simulink model "ssc_hydraulic_lift_LibLinks"  (R2025a)
settings: Solver=ode23t  StartTime=0.0  StopTime=20  MaxStep=0.02  RelTol=1e-3  AbsTol=1e-4  EnableMultiTasking=on
PreLoadFcn:
  | warning('off','Simulink:Commands:LoadMdlParameterizedLink');
PostLoadFcn:
  | warning off sm:compiler:topologyAnalysis:DanglingBlock
  | warning off Simulink:SL_SolverMaskedZC;
  | warning off Simulink:SL_SolverIgnoredZCBracketing;
  | warning off Simulink:Engine:SolverMinStepNonlinearIterWarnForDAE;
  | warning off simscape:compiler:sli:init:SolverNotRecommended
  | warning off Simulink:Engine:UsingDiscreteSolver
  | warning('off','sm:sli:setup:compile:LocalSolverNotSupported')
  | warning off physmod:simscape:compiler:sli:init:SolverNotRecommended
  | warning off sm:sli:visualization:ModelRefNotSupported
  | warning off Simulink:modelReference:ProtectedModelCallbackLostWarning
  | 
  | load_system('Cylinder_Lib');
  | load_system('Motor_Lib');
  | load_system('Valve_Lib');
  | load_system('Load_Lib');
StartFcn:
  | tic;
StopFcn:
  | Elapsed_Sim_Time = toc;
  | disp(['Elapsed Sim Time = ' num2str(Elapsed_Sim_Time)]);
undefined symbols (not defined in the file or in its folder): Scissor_Lift_Param, sigbuilder_block
libraries: fl_lib x4, nesl_utility x4, Cylinder_Lib x2, Controller_Lib x2, Load_Lib x2, Motor_Lib x2, Valve_Lib x2
Description:
  | Copyright 2015-2025 The MathWorks, Inc.
settings Model: ExtModeTrigDuration=500  Creator=smiller  LastModifiedBy=smiller
settings SolverCC: AutoScaleAbsTol=off  ConcurrentTasks=on  AlgebraicLoopSolver=TrustRegion  PositivePriorityOrder=on
settings DataIOCC: SaveFormat=Array  ReturnWorkspaceOutputs=off
settings OptimizationCC: BlockReduction=off  OptimizeBlockIOStorage=off  BufferReuse=off  ReuseModelBlockBuffer=off  GlobalBufferReuse=off  ExpressionFolding=off  ExpressionDepthLimit=2147483647.0  LocalBlockOutputs=off  ZeroExternalMemoryAtStartup=off  ZeroInternalMemoryAtStartup=off  OptimizeDataStoreBuffers=off  BusAssignmentInplaceUpdate=off
settings DebuggingCC: UnderspecifiedInitializationDetection=Classic  MergeDetectMultiDrivingBlocksExec=none  UnconnectedInputMsg=warning  UnconnectedOutputMsg=warning  UnconnectedLineMsg=warning  AllowSymbolicDim=off  StateNameClashWarn=warning  PregeneratedLibrarySubsystemCodeDiagnostic=none  SFUnexpectedBacktrackingDiag=warning  SFNoUnconditionalDefaultTransitionDiag=warning  SFExecutionAtInitializationDiag=none  ArithmeticOperatorsInVariantConditions=warning
settings ModelReferenceCC: EnableRefExpFcnMdlSchedulingChecks=on  PropagateSignalLabelsOutOfModel=off
settings SFSimCC: SimUseLocalCustomCode=off  CustomCodeUndefinedFunction=UseInterfaceOnly
settings RTWCC: RTWUseLocalCustomCode=off  Toolchain=Simulink Real-Time Toolchain  BuildConfiguration=Faster Runs  TargetLang=C++  GPUComputeCapability=3.5  DLArmComputeVersion=19.05
settings CodeAppCC: StateflowObjectComments=on
settings GRTTargetCC: TargetLangStandard=C++03 (ISO)  CodeInterfacePackaging=C++ class
settings ConfigComp: CovMetricSettings=dw  CovSaveCumulativeToWorkspaceVar=on  CovSaveSingleToWorkspaceVar=on  CovExternalEMLEnable=off  CovSFcnEnable=off
settings SimscapeCC: ExplicitSolverDiagnosticOptions=none  SimscapeNormalizeSystem=off  SimscapeNominalValues="[{\"value\":\"10\",\"unit\":\"V\"},{\"value\":\"1\",\"unit\":\"A\"},{\"value\":\"10\",\"unit\":\"N*m\"},{\"value\":\"10\",\"unit\":\"bar\"},{\"value\":\"100\",\"unit\":\"kJ/kg\"},{\"value\":\"1\",\"unit\":\"kW\"},{\"value\":\"300\",\"unit\":\"K\"},{\"value\":\"100\",\"unit\":\"cm^3/s\"},{\"value\":\"1\",\"unit\":\"kN\"},{\"value\":\"1\",\"unit\":\"g/cm^3\"},{\"value\":\"1\",\"unit\":\"l\"},{\"value\":\"1\",\"unit\":\"cm^2\"},{\"value\":\"60\",\"unit\":\"Hz\"}]"  SimscapeLogType=all  SimscapeLogSimulationStatistics=on  SimscapeLogName=simlog_ssc_hydraulic_lift  SimscapeLogLimitData=off
settings DiagnosticsConfigSet: SimMechanicsUnconnectedFramePorts=none  SimMechanicsConflictingReferenceFrames=none

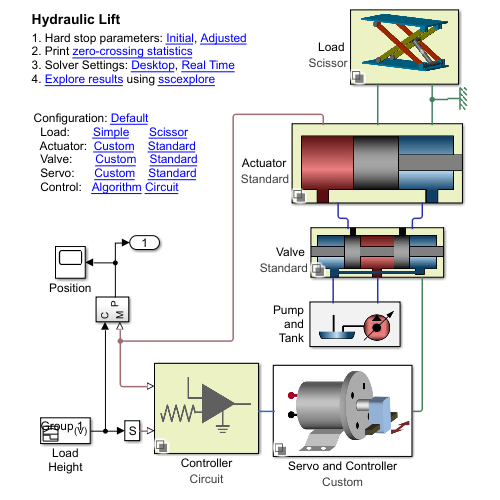
[thumbnail: Simulink's stored preview of the top-level diagram]
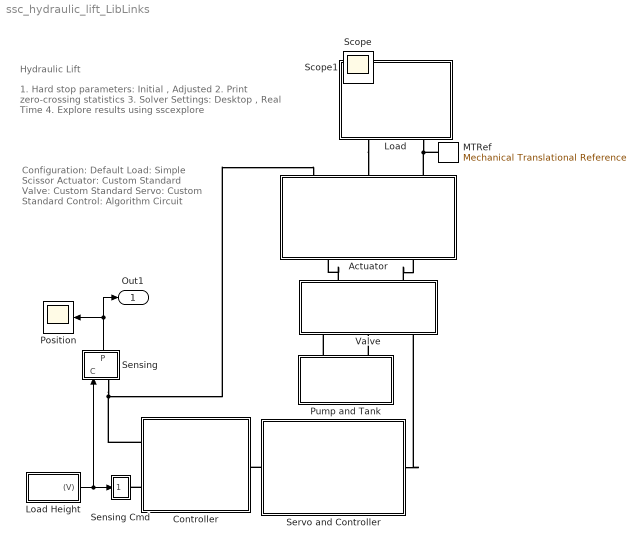
== system ssc_hydraulic_lift_LibLinks ==
  note: Hydraulic Lift
  note: 1. Hard stop parameters: Initial , Adjusted
      | 2. Print zero-crossing statistics
      | 3. Solver Settings: Desktop , Real Time
      | 4. Explore results using sscexplore
  note: Configuration: Default
      | Load: Simple Scissor
      | Actuator: Custom Standard
      | Valve: Custom Standard
      | Servo: Custom Standard
      | Control: Algorithm Circuit
  Actuator : Subsystem  Variant=on  VariantControlMode=label  LabelModeActiveChoice=Standard
      settings: AttributesFormatString=%<ActiveVariant>
      mask Display:
      | blk = ssc_hydraulic_lift_activeVariantBlock(gcb);
      | eval(get_param(blk, 'MaskDisplay'));
  Controller : Subsystem  Variant=on  VariantControlMode=label  LabelModeActiveChoice=Circuit
      settings: AttributesFormatString=%<ActiveVariant>
      mask Display:
      | blk = ssc_hydraulic_lift_activeVariantBlock(gcb);
      | eval(get_param(blk, 'MaskDisplay'));
  Load : Subsystem  Variant=on  VariantControlMode=label  LabelModeActiveChoice=Scissor
      settings: AttributesFormatString=%<ActiveVariant>
      mask Display:
      | blk = ssc_hydraulic_lift_activeVariantBlock(gcb);
      | eval(get_param(blk, 'MaskDisplay'));
  Load Height : Subsystem  Tag=STV Subsys  LoadFcn=sigbuilder_block('load');  StartFcn=sigbuilder_block('start');  StopFcn=sigbuilder_block('stop');  ClipboardFcn=sigbuilder_block('clipboard');  mask(Sigbuilder block){tuvar=[0:10]}
      mask help: Sigbuilder GUI
      mask init:
      | if ~strcmp(get_param(bdroot(gcbh),'SimulationStatus'),'stopped') tuvar = sigbuilder_block('maskInit'); end
      settings: CopyFcn=sigbuilder_block('copy');  DeleteFcn=sigbuilder_block('delete');  ModelCloseFcn=sigbuilder_block('modelClose');  PreSaveFcn=sigbuilder_block('preSave');  PauseFcn=sigbuilder_block('pause')  ContinueFcn=sigbuilder_block('continue')  NameChangeFcn=sigbuilder_block('namechange');  OpenFcn=sigbuilder_block('open',[109.2 227.4 330.6 249.6 ]);  CloseFcn=sigbuilder_block('close');
      mask Display: plot(0, 0, 100, 100,[2, 2, 32, 32, 2], [68, 8, 8, 68, 68],[32, 2], [38, 38], [32, 19, 2],[53, 60, 44], [32, 17, 17, 2],[16, 16, 31, 31]);txt = getActiveGroup(gcbh);text(2, 100, txt,'verticalAlignment', 'top');
  MTRef : fl_lib/Mechanical/Translational Elements/Mechanical Translational Reference
  Position : Scope
      settings: ActiveDisplayYMinimum=-79.32809  ActiveDisplayYMaximum=179.34288  DataLoggingVariableName=LoadPosition_DATA
  Pump and Tank : Subsystem
      mask Display: image('Pump_IMAGE.jpg');
  Sensing : Subsystem
  Sensing Cmd : Subsystem
      mask Display: disp('S')
  Servo and Controller : Subsystem  Variant=on  VariantControlMode=label  LabelModeActiveChoice=Custom
      settings: AttributesFormatString=%<ActiveVariant>
      mask Display:
      | blk = ssc_hydraulic_lift_activeVariantBlock(gcb);
      | eval(get_param(blk, 'MaskDisplay'));
  Valve : Subsystem  Variant=on  VariantControlMode=label  LabelModeActiveChoice=Standard
      settings: AttributesFormatString=%<ActiveVariant>
      mask Display:
      | blk = ssc_hydraulic_lift_activeVariantBlock(gcb);
      | eval(get_param(blk, 'MaskDisplay'));
  Out1 : Outport  VectorParamsAs1DForOutWhenUnconnected=off
  Scope : Scope
      settings: ActiveDisplayYMinimum=-0.84217  ActiveDisplayYMaximum=5.75412
  Scope1 : Scope
      settings: ActiveDisplayYMinimum=-0.31315  ActiveDisplayYMaximum=0.39292  DataLoggingVariableName=ScopeData2
  wires:
  Load Height/1((V)) -> Sensing/1(C), Sensing Cmd/1(In1)
  Sensing/1(P) -> Position/1, Out1/1
  connections:
  MTRef/LConn1 -- Load/LConn2 -- Actuator/RConn3
  Valve/RConn1 -- Actuator/LConn1
  Valve/RConn2 -- Actuator/LConn2
  Controller/LConn1 -- Sensing/LConn1 -- Actuator/RConn1
  Load/LConn1 -- Actuator/RConn2
  Servo and Controller/RConn1 -- Valve/LConn3
  Servo and Controller/LConn1 -- Controller/RConn1
  Controller/LConn2 -- Sensing Cmd/RConn1
  Pump and Tank/RConn1 -- Valve/LConn1
  Pump and Tank/RConn2 -- Valve/LConn2

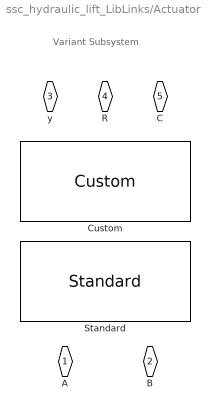
== system ssc_hydraulic_lift_LibLinks/Actuator ==
  note: Variant Subsystem
  Custom : Cylinder_Lib/Custom  VariantControl=Custom  A=5e-4  V=10e-6  PA=200  PB=0  T=200  hs_k=actuator_hs_k  hs_b=actuator_hs_b
  Standard : Cylinder_Lib/Standard  VariantControl=Standard  A=5e-4  V=10e-6  PA=200  PB=0  T=200  hs_k=actuator_hs_k  hs_b=actuator_hs_b
  A : PMIOPort  Side=Left
  B : PMIOPort  Port=2  Side=Left
  y : PMIOPort  Port=3  Side=Right
  R : PMIOPort  Port=4  Side=Right
  C : PMIOPort  Port=5  Side=Right

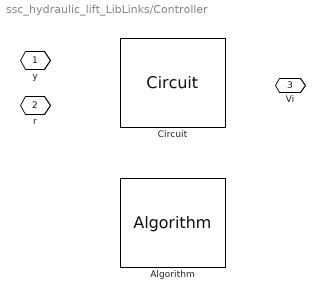
== system ssc_hydraulic_lift_LibLinks/Controller ==
  Algorithm : Controller_Lib/Algorithm  SystemSampleTime=-1  VariantControl=Algorithm  VariantActivationTime=update diagram  EmptyChoice=off  PassThrough=off  PassThroughVariantControl=(default)  EmptyChoiceVariantControl=(default)  AllowFlexibleInterface=on  Latency=0  AutoFrameSizeCalculation=off
  Circuit : Controller_Lib/Circuit  SystemSampleTime=-1  VariantControl=Circuit  VariantActivationTime=update diagram  EmptyChoice=off  PassThrough=off  PassThroughVariantControl=(default)  EmptyChoiceVariantControl=(default)  AllowFlexibleInterface=on  Latency=0  AutoFrameSizeCalculation=off
  y : PMIOPort  Tag=PMCPort  Side=Left
  r : PMIOPort  Tag=PMCPort  Port=2  Side=Left
  Vi : PMIOPort  Port=3  Side=Right

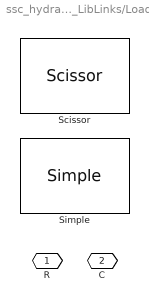
== system ssc_hydraulic_lift_LibLinks/Load ==
  Scissor : Load_Lib/Scissor  SystemSampleTime=-1  VariantControl=Scissor  VariantActivationTime=update diagram  EmptyChoice=off  PassThrough=off  PassThroughVariantControl=(default)  EmptyChoiceVariantControl=(default)  AllowFlexibleInterface=on  Latency=0  AutoFrameSizeCalculation=off
  Simple : Load_Lib/Simple  SystemSampleTime=-1  VariantControl=Simple  VariantActivationTime=update diagram  EmptyChoice=off  PassThrough=off  PassThroughVariantControl=(default)  EmptyChoiceVariantControl=(default)  AllowFlexibleInterface=on  Latency=0  AutoFrameSizeCalculation=off
  R : PMIOPort  Side=Left
  C : PMIOPort  Port=2  Side=Left

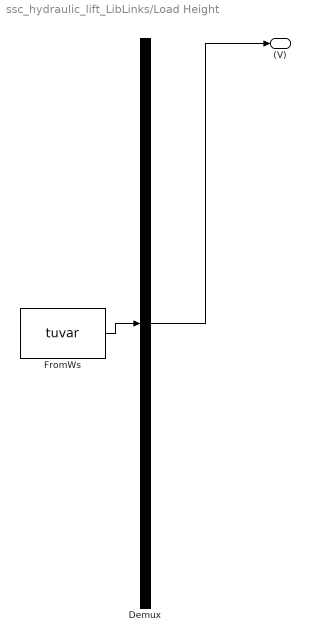
== system ssc_hydraulic_lift_LibLinks/Load Height ==
  Demux : Demux  Tag=STV Demux  Outputs=1
      settings: DisplayOption=none
  FromWs : FromWorkspace  Tag=STV FromWs  VariableName=tuvar
      SigBuilderData=|
      | common.afterFinalStr = 'Extrapolate'
      | common.sampleTime = 0
      | dataSet.timeRange = [0 20]
      | dataSet.name = 'Group 1'
      | sbobj.Groups.Name = 'Group 1'
      | sbobj.Groups.Signals.Name = '(V)'
      | sbobj.Groups.Signals.XData = [0 1 3 4 10 12 15 20]
      | sbobj.Groups.Signals.YData = [2.5 2.5 5 5 0 0 2.5 2.5]
      | sbobj.Groups.TimeRange = [0 20]
  (V) : Outport  Tag=STV Outport  VectorParamsAs1DForOutWhenUnconnected=off
  wires:
  Demux/1 -> (V)/1
  FromWs/1 -> Demux/1

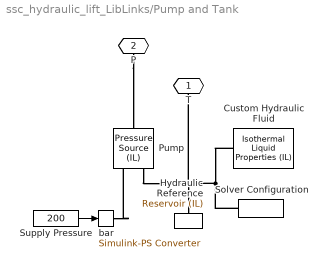
== system ssc_hydraulic_lift_LibLinks/Pump and Tank ==
  Custom Hydraulic Fluid : fl_lib/Isothermal Liquid/Utilities/Isothermal Liquid Properties (IL)  rho_L_atm=850 kg/m^3  bulk_modulus_model=foundation.enum.bulk_modulus_model.const  beta_gain=6  beta_L_atm=8e+08 Pa  nu_atm=1.8e-05 m^2/s  p_atm=0.101325 MPa  p_min=1 Pa  properties_range_check=simscape.enum.assert.action.error  air_fraction=0.005  polytropic_index=1.0  rho_g_atm=1.225 kg/m^3  air_dissolution_model=false  p_crit=3 MPa
      settings: LibrarySourceBlock=fl_lib/Isothermal Liquid/Utilities/Isothermal Liquid Properties (IL)
  Hydraulic Reference : fl_lib/Isothermal Liquid/Elements/Reservoir (IL)  reservoir_type=foundation.enum.constant_controlled.constant  pressure_spec=foundation.enum.pressure_spec.atmospheric  reservoir_pressure=0.101325 MPa
  Pump : fl_lib/Isothermal Liquid/Sources/Pressure Source (IL)  source_type=foundation.enum.constant_controlled.controlled  pressure_differential=0 MPa
      settings: InternalSimscapePortConfiguration="{\"Bottom\":[],\"Left\":[{\"id\":\"A\",\"label\":\"A\",\"type\":\"foundation.isothermal_liquid.isothermal_liquid\"},{\"id\":\"P\",\"label\":\"P\",\"type\":\"input\"}],\"Right\":[{\"id\":\"B\",\"label\":\"B\",\"type\":\"foundation.isothermal_liquid.isothermal_liquid\"}],\"Top\":[]}"
  Solver Configuration : nesl_utility/Solver Configuration  PhysicalDomain=network_engine_domain  SubClassName=solver  LeftPortType=input  RightPortType=generic  Tones=[]  Harmonics=[]  SimulateNoise=off  Profile=off  UseLocalSampling=off  EnableSwitchedLinearOptims=on  FrequencyDomain=off  UseCCode=off  RelTol=0.001  AbsTol=1e-06  MinStep=1e-09  ToWorkspace=off  RevertToSquareIcSolve=off  NumHomotopyIterations=100  PhasorMode=off  PhasorModeNumHarmonics=1  ConsistencySolver=NEWTON_FTOL  IndexReductionMethod=DerivativeReplacement  DoDC=off  ResidualTolerance=1e-9  ConsistencyTolSource=GLOBAL  ConsistencyAbsTol=0.001  ConsistencyRelTol=0.001  ConsistencyTolFactor=0.001  UseLocalSolver=off  LocalSolverChoice=NE_BACKWARD_EULER_ADVANCER  ResolveIndetEquations=on  FunctionEvalNumThread=1  LocalSolverSampleTime=0.002  DoFixedCost=off  MaxNonlinIter=4  MaxModeIter=2  ComputeImpulses=off  ImpulseIterations=2  LinearAlgebra=Sparse  LinearAlgebraNumThread=0  EquationFormulation=NE_TIME_EF  DelaysMemoryBudget=1024  AutomaticFiltering=on  FilteringTimeConstant=0.001  PartitionStorageMethod=AS_NEEDED  PartitionMemoryBudget=1024  PartitionMethod=FAST  MultibodyUseLocalSolver=off  MultibodyLocalSolverChoice=ODE1  MultibodyLocalSolverSampleTime=0.001
  Supply Pressure : Constant  Value=200
  bar : nesl_utility/Simulink-PS Converter  PhysicalDomain=network_engine_domain  SubClassName=ps_input  LeftPortType=input  RightPortType=output  PseudoPeriodic=off  Frequencies=[]  NoiseDistribution=none  NoiseParameters=[]  Unit=bar  AffineConversion=off  FilteringAndDerivatives=zero  SimscapeFilterOrder=1  InputFilterTimeConstant=0.005  UdotUserProvided=0
  T : PMIOPort  Side=Right
  P : PMIOPort  Port=2  Side=Right
  wires:
  Supply Pressure/1 -> bar/1
  connections:
  Custom Hydraulic Fluid/RConn1 -- Solver Configuration/RConn1 -- T/RConn1 -- Pump/LConn1 -- Hydraulic Reference/LConn1
  P/RConn1 -- Pump/RConn1
  bar/RConn1 -- Pump/LConn2

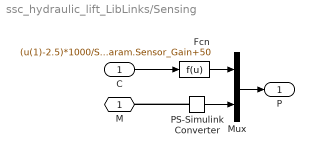
== system ssc_hydraulic_lift_LibLinks/Sensing ==
  C : Inport
  Fcn : Fcn  Expr=(u(1)-2.5)*1000/Scissor_Lift_Param.Sensor_Gain+50
  Mux : Mux  Inputs=2
  PS-Simulink Converter : nesl_utility/PS-Simulink Converter  PhysicalDomain=network_engine_domain  SubClassName=ps_output  LeftPortType=input  RightPortType=output  PseudoPeriodic=off  Frequencies=[]  VectorFormat=1-D array  Unit=mm  AffineConversion=off
  M : PMIOPort  Side=Left
  P : Outport  VectorParamsAs1DForOutWhenUnconnected=off
  wires:
  PS-Simulink Converter/1 -> Mux/2
  Mux/1 -> P/1
  Fcn/1 -> Mux/1
  C/1 -> Fcn/1
  connections:
  PS-Simulink Converter/LConn1 -- M/RConn1

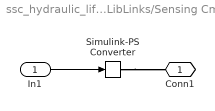
== system ssc_hydraulic_lift_LibLinks/Sensing Cmd ==
  In1 : Inport
  Simulink-PS Converter : nesl_utility/Simulink-PS Converter  PhysicalDomain=network_engine_domain  SubClassName=ps_input  LeftPortType=input  RightPortType=output  PseudoPeriodic=off  Frequencies=[]  NoiseDistribution=none  NoiseParameters=[]  Unit=V  AffineConversion=off  FilteringAndDerivatives=filter  SimscapeFilterOrder=1  InputFilterTimeConstant=0.005  UdotUserProvided=1
  Conn1 : PMIOPort  Side=Right
  wires:
  In1/1 -> Simulink-PS Converter/1
  connections:
  Simulink-PS Converter/RConn1 -- Conn1/RConn1

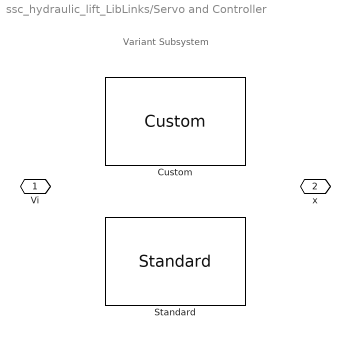
== system ssc_hydraulic_lift_LibLinks/Servo and Controller ==
  note: Variant Subsystem
  Custom : Motor_Lib/Custom  VariantControl=Custom  G=0.5e-3/(pi/2)  x_max=0.5  J=1e-4  lambda=motor_damping  R=10  L=2.5  Kt=0.04  R_controller=[10e3 10e3 10e3 100e3 50 100e3 10e3]
  Standard : Motor_Lib/Standard  VariantControl=Standard  G=0.5e-3/(pi/2)  x_max=0.5  J=1e-4  lambda=motor_damping  R=10  L=2.5  Kt=0.04  R_controller=[10e3 10e3 10e3 100e3 50 100e3 10e3]
  Vi : PMIOPort  Side=Left
  x : PMIOPort  Port=2  Side=Right

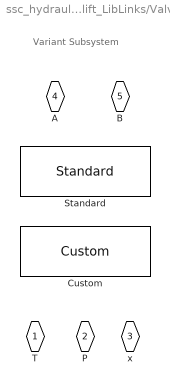
== system ssc_hydraulic_lift_LibLinks/Valve ==
  note: Variant Subsystem
  Custom : Valve_Lib/Custom  VariantControl=Custom  K_V=0.5  x_max=0.5  A_max=9  x_lap=0.02  A_leak=0.25
  Standard : Valve_Lib/Standard  VariantControl=Standard  K_V=0.5  x_max=0.5  A_max=9  x_lap=0.02  A_leak=0.25
  T : PMIOPort  Tag=PMCPort  Side=Left
  P : PMIOPort  Tag=PMCPort  Port=2  Side=Left
  x : PMIOPort  Tag=PMCPort  Port=3  Side=Left
  A : PMIOPort  Tag=PMCPort  Port=4  Side=Right
  B : PMIOPort  Tag=PMCPort  Port=5  Side=Right
